simulink model "ASM_Traffic_MultiCore"  (R2026a)
settings: Solver=ode1  StartTime=SIM.tstart.v  StopTime=SIM.tend.v  FixedStep=SIM.StepSize.v
PostLoadFcn:
  | if any(exist('dsrtsu_mdlpostloadfcn', 'file') ~= 0), dsrtsu_mdlpostloadfcn('Execute', bdroot); end
  | try, asm_mdl_postloadfcn(bdroot, 'UpdateModel', 3600); catch, disp(lasterr); end,
InitFcn:
  | , if any(exist('rtifpga_mdlclblib', 'file') ~= 0), rtifpga_mdlclblib('Init', bdroot); end,
  | , if any(exist('dsmpb_private', 'file') ~= 0), dsmpb_private('dsmpb_mdlclblib', 'Init', bdroot); end,
model workspace (MAT data in the model file):
  asmReferencePath = [0 0.01 0.02 0.03 0.04 0.05 0.06 0.07 0.08 0.09 0.1 0.11 ... (350007 elements, 50001x7)]
  roadBounds : Simulink.Parameter (value not decoded)
  safetyAxes : Simulink.Parameter (value not decoded)
undefined symbols (not defined in the file): _to_, a0b2, ASM_BrakeHydraulics_DemoSystems, ASM_VehicleDynamics_DemoSystems, b98103fe8ad365046cd0, BrakeCircuit, controllerConfig, CPT, Crankshaft, DiscIntNeverNeededParam, dsmsi, FinalDriveAssembly, MDL, ModeSignals, mu, Pos_BrakePedal_Maneuver, rad, RefSignals, roadFamilyData, roadFamilyId, s_to_rpm, SIM, SoftECU, Suspension, Tire, Transmission
libraries: ASM_Traffic_lib x135, simulink x98, ASM_Utils_lib x77, ASM_VehicleDynamics_lib x70, ASM_Environment_lib x22, dsmpblib x20, dsmsilib x15, MDLD_Utils_lib x10, ASM_BrakeHydraulics_lib x3, sl_discontinuities x2
(part 57 of 65)

== system ASM_Traffic_MultiCore/Environment/GroundTruth/UserInterface/PAR_Plant/Fellow_Vehicles/Lightstates_Fellow3/Indicator_State[] ==
  Fellow_TurnLights[] : Inport
  ASM_OSI_Mapping : Subsystem
  Ext_Indicator_State[] : Constant  Value=0
  Multiport Switch : MultiPortSwitch  DataPortOrder=Zero-based contiguous  zeroidx=on  SaturateOnIntegerOverflow=off  InputSameDT=off
  Rounding Function : Rounding  Operator=round
  Saturation : Saturate  UpperLimit=2  LowerLimit=0
  Stim_Indicator_State[] : Constant  Value=0
  Sw_Indicator[0Stim|1Ext|2Mnv] : Constant  Value=2
  Indicator_State[] : Outport  VectorParamsAs1DForOutWhenUnconnected=off
  wires:
  ASM_OSI_Mapping/1(Indicator_State[]) -> Multiport Switch/4  "Mnv_Indicator_State[]"
  Stim_Indicator_State[]/1 -> Multiport Switch/2  "Stim_Indicator_State[]"
  Multiport Switch/1 -> Indicator_State[]/1  "Indicator_State[]"
  Saturation/1 -> Multiport Switch/1
  Rounding Function/1 -> Saturation/1
  Ext_Indicator_State[]/1 -> Multiport Switch/3  "Ext_Indicator_State[]"
  Fellow_TurnLights[]/1 -> ASM_OSI_Mapping/1(Fellow_TurnLights[])
  Sw_Indicator[0Stim|1Ext|2Mnv]/1 -> Rounding Function/1  "Sw_Indicator[0Stim|1Ext|2Mnv]"

== system ASM_Traffic_MultiCore/Environment/GroundTruth/UserInterface/PAR_Plant/Fellow_Vehicles/Lightstates_Fellow30/Indicator_State[] ==
  Fellow_TurnLights[] : Inport
  ASM_OSI_Mapping : Subsystem
  Ext_Indicator_State[] : Constant  Value=0
  Multiport Switch : MultiPortSwitch  DataPortOrder=Zero-based contiguous  zeroidx=on  SaturateOnIntegerOverflow=off  InputSameDT=off
  Rounding Function : Rounding  Operator=round
  Saturation : Saturate  UpperLimit=2  LowerLimit=0
  Stim_Indicator_State[] : Constant  Value=0
  Sw_Indicator[0Stim|1Ext|2Mnv] : Constant  Value=2
  Indicator_State[] : Outport  VectorParamsAs1DForOutWhenUnconnected=off
  wires:
  Sw_Indicator[0Stim|1Ext|2Mnv]/1 -> Rounding Function/1  "Sw_Indicator[0Stim|1Ext|2Mnv]"
  Fellow_TurnLights[]/1 -> ASM_OSI_Mapping/1(Fellow_TurnLights[])
  Ext_Indicator_State[]/1 -> Multiport Switch/3  "Ext_Indicator_State[]"
  Rounding Function/1 -> Saturation/1
  Saturation/1 -> Multiport Switch/1
  Multiport Switch/1 -> Indicator_State[]/1  "Indicator_State[]"
  Stim_Indicator_State[]/1 -> Multiport Switch/2  "Stim_Indicator_State[]"
  ASM_OSI_Mapping/1(Indicator_State[]) -> Multiport Switch/4  "Mnv_Indicator_State[]"

== system ASM_Traffic_MultiCore/Environment/GroundTruth/UserInterface/PAR_Plant/Fellow_Vehicles/Lightstates_Fellow4/Indicator_State[] ==
  Fellow_TurnLights[] : Inport
  ASM_OSI_Mapping : Subsystem
  Ext_Indicator_State[] : Constant  Value=0
  Multiport Switch : MultiPortSwitch  DataPortOrder=Zero-based contiguous  zeroidx=on  SaturateOnIntegerOverflow=off  InputSameDT=off
  Rounding Function : Rounding  Operator=round
  Saturation : Saturate  UpperLimit=2  LowerLimit=0
  Stim_Indicator_State[] : Constant  Value=0
  Sw_Indicator[0Stim|1Ext|2Mnv] : Constant  Value=2
  Indicator_State[] : Outport  VectorParamsAs1DForOutWhenUnconnected=off
  wires:
  Sw_Indicator[0Stim|1Ext|2Mnv]/1 -> Rounding Function/1  "Sw_Indicator[0Stim|1Ext|2Mnv]"
  Fellow_TurnLights[]/1 -> ASM_OSI_Mapping/1(Fellow_TurnLights[])
  Ext_Indicator_State[]/1 -> Multiport Switch/3  "Ext_Indicator_State[]"
  Rounding Function/1 -> Saturation/1
  Saturation/1 -> Multiport Switch/1
  Multiport Switch/1 -> Indicator_State[]/1  "Indicator_State[]"
  Stim_Indicator_State[]/1 -> Multiport Switch/2  "Stim_Indicator_State[]"
  ASM_OSI_Mapping/1(Indicator_State[]) -> Multiport Switch/4  "Mnv_Indicator_State[]"

== system ASM_Traffic_MultiCore/Environment/GroundTruth/UserInterface/PAR_Plant/Fellow_Vehicles/Lightstates_Fellow5/Indicator_State[] ==
  Fellow_TurnLights[] : Inport
  ASM_OSI_Mapping : Subsystem
  Ext_Indicator_State[] : Constant  Value=0
  Multiport Switch : MultiPortSwitch  DataPortOrder=Zero-based contiguous  zeroidx=on  SaturateOnIntegerOverflow=off  InputSameDT=off
  Rounding Function : Rounding  Operator=round
  Saturation : Saturate  UpperLimit=2  LowerLimit=0
  Stim_Indicator_State[] : Constant  Value=0
  Sw_Indicator[0Stim|1Ext|2Mnv] : Constant  Value=2
  Indicator_State[] : Outport  VectorParamsAs1DForOutWhenUnconnected=off
  wires:
  ASM_OSI_Mapping/1(Indicator_State[]) -> Multiport Switch/4  "Mnv_Indicator_State[]"
  Stim_Indicator_State[]/1 -> Multiport Switch/2  "Stim_Indicator_State[]"
  Multiport Switch/1 -> Indicator_State[]/1  "Indicator_State[]"
  Saturation/1 -> Multiport Switch/1
  Rounding Function/1 -> Saturation/1
  Ext_Indicator_State[]/1 -> Multiport Switch/3  "Ext_Indicator_State[]"
  Fellow_TurnLights[]/1 -> ASM_OSI_Mapping/1(Fellow_TurnLights[])
  Sw_Indicator[0Stim|1Ext|2Mnv]/1 -> Rounding Function/1  "Sw_Indicator[0Stim|1Ext|2Mnv]"

== system ASM_Traffic_MultiCore/Environment/GroundTruth/UserInterface/PAR_Plant/Fellow_Vehicles/Lightstates_Fellow6/Indicator_State[] ==
  Fellow_TurnLights[] : Inport
  ASM_OSI_Mapping : Subsystem
  Ext_Indicator_State[] : Constant  Value=0
  Multiport Switch : MultiPortSwitch  DataPortOrder=Zero-based contiguous  zeroidx=on  SaturateOnIntegerOverflow=off  InputSameDT=off
  Rounding Function : Rounding  Operator=round
  Saturation : Saturate  UpperLimit=2  LowerLimit=0
  Stim_Indicator_State[] : Constant  Value=0
  Sw_Indicator[0Stim|1Ext|2Mnv] : Constant  Value=2
  Indicator_State[] : Outport  VectorParamsAs1DForOutWhenUnconnected=off
  wires:
  Sw_Indicator[0Stim|1Ext|2Mnv]/1 -> Rounding Function/1  "Sw_Indicator[0Stim|1Ext|2Mnv]"
  Fellow_TurnLights[]/1 -> ASM_OSI_Mapping/1(Fellow_TurnLights[])
  Ext_Indicator_State[]/1 -> Multiport Switch/3  "Ext_Indicator_State[]"
  Rounding Function/1 -> Saturation/1
  Saturation/1 -> Multiport Switch/1
  Multiport Switch/1 -> Indicator_State[]/1  "Indicator_State[]"
  Stim_Indicator_State[]/1 -> Multiport Switch/2  "Stim_Indicator_State[]"
  ASM_OSI_Mapping/1(Indicator_State[]) -> Multiport Switch/4  "Mnv_Indicator_State[]"

== system ASM_Traffic_MultiCore/Environment/GroundTruth/UserInterface/PAR_Plant/Fellow_Vehicles/Lightstates_Fellow7/Indicator_State[] ==
  Fellow_TurnLights[] : Inport
  ASM_OSI_Mapping : Subsystem
  Ext_Indicator_State[] : Constant  Value=0
  Multiport Switch : MultiPortSwitch  DataPortOrder=Zero-based contiguous  zeroidx=on  SaturateOnIntegerOverflow=off  InputSameDT=off
  Rounding Function : Rounding  Operator=round
  Saturation : Saturate  UpperLimit=2  LowerLimit=0
  Stim_Indicator_State[] : Constant  Value=0
  Sw_Indicator[0Stim|1Ext|2Mnv] : Constant  Value=2
  Indicator_State[] : Outport  VectorParamsAs1DForOutWhenUnconnected=off
  wires:
  ASM_OSI_Mapping/1(Indicator_State[]) -> Multiport Switch/4  "Mnv_Indicator_State[]"
  Stim_Indicator_State[]/1 -> Multiport Switch/2  "Stim_Indicator_State[]"
  Multiport Switch/1 -> Indicator_State[]/1  "Indicator_State[]"
  Saturation/1 -> Multiport Switch/1
  Rounding Function/1 -> Saturation/1
  Ext_Indicator_State[]/1 -> Multiport Switch/3  "Ext_Indicator_State[]"
  Fellow_TurnLights[]/1 -> ASM_OSI_Mapping/1(Fellow_TurnLights[])
  Sw_Indicator[0Stim|1Ext|2Mnv]/1 -> Rounding Function/1  "Sw_Indicator[0Stim|1Ext|2Mnv]"

== system ASM_Traffic_MultiCore/Environment/GroundTruth/UserInterface/PAR_Plant/Fellow_Vehicles/Lightstates_Fellow8/Indicator_State[] ==
  Fellow_TurnLights[] : Inport
  ASM_OSI_Mapping : Subsystem
  Ext_Indicator_State[] : Constant  Value=0
  Multiport Switch : MultiPortSwitch  DataPortOrder=Zero-based contiguous  zeroidx=on  SaturateOnIntegerOverflow=off  InputSameDT=off
  Rounding Function : Rounding  Operator=round
  Saturation : Saturate  UpperLimit=2  LowerLimit=0
  Stim_Indicator_State[] : Constant  Value=0
  Sw_Indicator[0Stim|1Ext|2Mnv] : Constant  Value=2
  Indicator_State[] : Outport  VectorParamsAs1DForOutWhenUnconnected=off
  wires:
  Sw_Indicator[0Stim|1Ext|2Mnv]/1 -> Rounding Function/1  "Sw_Indicator[0Stim|1Ext|2Mnv]"
  Fellow_TurnLights[]/1 -> ASM_OSI_Mapping/1(Fellow_TurnLights[])
  Ext_Indicator_State[]/1 -> Multiport Switch/3  "Ext_Indicator_State[]"
  Rounding Function/1 -> Saturation/1
  Saturation/1 -> Multiport Switch/1
  Multiport Switch/1 -> Indicator_State[]/1  "Indicator_State[]"
  Stim_Indicator_State[]/1 -> Multiport Switch/2  "Stim_Indicator_State[]"
  ASM_OSI_Mapping/1(Indicator_State[]) -> Multiport Switch/4  "Mnv_Indicator_State[]"

== system ASM_Traffic_MultiCore/Environment/GroundTruth/UserInterface/PAR_Plant/Fellow_Vehicles/Lightstates_Fellow9/Indicator_State[] ==
  Fellow_TurnLights[] : Inport
  ASM_OSI_Mapping : Subsystem
  Ext_Indicator_State[] : Constant  Value=0
  Multiport Switch : MultiPortSwitch  DataPortOrder=Zero-based contiguous  zeroidx=on  SaturateOnIntegerOverflow=off  InputSameDT=off
  Rounding Function : Rounding  Operator=round
  Saturation : Saturate  UpperLimit=2  LowerLimit=0
  Stim_Indicator_State[] : Constant  Value=0
  Sw_Indicator[0Stim|1Ext|2Mnv] : Constant  Value=2
  Indicator_State[] : Outport  VectorParamsAs1DForOutWhenUnconnected=off
  wires:
  ASM_OSI_Mapping/1(Indicator_State[]) -> Multiport Switch/4  "Mnv_Indicator_State[]"
  Stim_Indicator_State[]/1 -> Multiport Switch/2  "Stim_Indicator_State[]"
  Multiport Switch/1 -> Indicator_State[]/1  "Indicator_State[]"
  Saturation/1 -> Multiport Switch/1
  Rounding Function/1 -> Saturation/1
  Ext_Indicator_State[]/1 -> Multiport Switch/3  "Ext_Indicator_State[]"
  Fellow_TurnLights[]/1 -> ASM_OSI_Mapping/1(Fellow_TurnLights[])
  Sw_Indicator[0Stim|1Ext|2Mnv]/1 -> Rounding Function/1  "Sw_Indicator[0Stim|1Ext|2Mnv]"

== system ASM_Traffic_MultiCore/Environment/GroundTruth/UserInterface/PAR_Plant/HostVehicle_Data_AutomatedDrivingFunction/AutomatedDrivingFunction_1/Mappings ==
  Driver_Override_ACC_Active_In[0Off|1On] : Inport
  Driver_Override_ACC_Reason[0NoOverride|1BrakePedal|2AccPedal] : Inport  Port=2
  ACC_State[1OFF|2Standby|3ON] : Inport  Port=3
  Compare To Constant : simulink/Logic and Bit Operations/Compare To Constant  relop===  const=1  OutDataTypeStr=boolean
  Data Type Conversion : DataTypeConversion  SaturateOnIntegerOverflow=off  RndMeth=Floor
  DriverOverride_Reason_Idx[0BrakePedal|1SteeringInput] : Constant  Value=0
  Multiport Switch1 : MultiPortSwitch  DataPortIndices={-2,-1,0,1,2,3}  DataPortForDefault=Additional data port  DiagnosticForDefault=None  SaturateOnIntegerOverflow=off  InputSameDT=off
  Off : Constant  Value=0
  State_Active : Constant  Value=6
  State_Available : Constant  Value=4
  State_Other : Constant
  State_Standby : Constant  Value=5
  Switch1 : Switch  Criteria=u2 > Threshold  SaturateOnIntegerOverflow=off  InputSameDT=off
  Driver_Override_ACC_Active[0Off|1On] : Outport
  DriverOverride_Reason_Idx[] : Outport  Port=2
  State_Idx[] : Outport  Port=3
  wires:
  Driver_Override_ACC_Reason[0NoOverride|1BrakePedal|2AccPedal]/1 -> Compare To Constant/1
  Compare To Constant/1 -> Switch1/2
  ACC_State[1OFF|2Standby|3ON]/1 -> Multiport Switch1/1
  Multiport Switch1/1 -> State_Idx[]/1
  State_Standby/1 -> Multiport Switch1/3
  State_Available/1 -> Multiport Switch1/2
  State_Active/1 -> Multiport Switch1/4
  State_Other/1 -> Multiport Switch1/5
  Driver_Override_ACC_Active_In[0Off|1On]/1 -> Data Type Conversion/1
  Data Type Conversion/1 -> Switch1/1
  Off/1 -> Switch1/3
  Switch1/1 -> Driver_Override_ACC_Active[0Off|1On]/1
  DriverOverride_Reason_Idx[0BrakePedal|1SteeringInput]/1 -> DriverOverride_Reason_Idx[]/1

== system ASM_Traffic_MultiCore/Environment/GroundTruth/UserInterface/PAR_Plant/HostVehicle_Data_AutomatedDrivingFunction/AutomatedDrivingFunction_2/Mappings ==
  Driver_Override_ACC_Active_In[0Off|1On] : Inport
  Driver_Override_ACC_Reason[0NoOverride|1BrakePedal|2AccPedal] : Inport  Port=2
  AEB[0|1] : Inport  Port=3
  Compare To Constant : simulink/Logic and Bit Operations/Compare To Constant  relop===  const=1  OutDataTypeStr=boolean
  Data Type Conversion : DataTypeConversion  SaturateOnIntegerOverflow=off  RndMeth=Floor
  DriverOverride_Reason_Idx[0BrakePedal|1SteeringInput] : Constant  Value=0
  Multiport Switch1 : MultiPortSwitch  DataPortOrder=Zero-based contiguous  Inputs=2  DataPortIndices={-2,-1,0,1,2,3}  DataPortForDefault=Additional data port  DiagnosticForDefault=None  zeroidx=on  SaturateOnIntegerOverflow=off  InputSameDT=off
  Off : Constant  Value=0
  State_Active : Constant  Value=6
  State_Available : Constant  Value=4
  State_Other : Constant
  Switch1 : Switch  Criteria=u2 > Threshold  SaturateOnIntegerOverflow=off  InputSameDT=off
  Driver_Override_ACC_Active[0Off|1On] : Outport
  DriverOverride_Reason_Idx[] : Outport  Port=2
  State_Idx[] : Outport  Port=3
  wires:
  DriverOverride_Reason_Idx[0BrakePedal|1SteeringInput]/1 -> DriverOverride_Reason_Idx[]/1
  Driver_Override_ACC_Reason[0NoOverride|1BrakePedal|2AccPedal]/1 -> Compare To Constant/1
  AEB[0|1]/1 -> Multiport Switch1/1
  Multiport Switch1/1 -> State_Idx[]/1
  State_Active/1 -> Multiport Switch1/3
  State_Available/1 -> Multiport Switch1/2
  State_Other/1 -> Multiport Switch1/4
  Driver_Override_ACC_Active_In[0Off|1On]/1 -> Data Type Conversion/1
  Off/1 -> Switch1/3
  Compare To Constant/1 -> Switch1/2
  Data Type Conversion/1 -> Switch1/1
  Switch1/1 -> Driver_Override_ACC_Active[0Off|1On]/1

== system ASM_Traffic_MultiCore/Environment/GroundTruth/UserInterface/PAR_Plant/HostVehicle_Data_AutomatedDrivingFunction/AutomatedDrivingFunction_3/Mappings ==
  Driver_Override_ACC_Active_In[0Off|1On] : Inport
  Driver_Override_ACC_Reason[0NoOverride|1BrakePedal|2AccPedal] : Inport  Port=2
  FCW[0|1] : Inport  Port=3
  Compare To Constant : simulink/Logic and Bit Operations/Compare To Constant  relop===  const=1  OutDataTypeStr=boolean
  Data Type Conversion : DataTypeConversion  SaturateOnIntegerOverflow=off  RndMeth=Floor
  DriverOverride_Reason_Idx[0BrakePedal|1SteeringInput] : Constant  Value=0
  Multiport Switch1 : MultiPortSwitch  DataPortOrder=Zero-based contiguous  Inputs=2  DataPortIndices={-2,-1,0,1,2,3}  DataPortForDefault=Additional data port  DiagnosticForDefault=None  zeroidx=on  SaturateOnIntegerOverflow=off  InputSameDT=off
  Off : Constant  Value=0
  State_Active : Constant  Value=6
  State_Available : Constant  Value=4
  State_Other : Constant
  Switch1 : Switch  Criteria=u2 > Threshold  SaturateOnIntegerOverflow=off  InputSameDT=off
  Driver_Override_ACC_Active[0Off|1On] : Outport
  DriverOverride_Reason_Idx[] : Outport  Port=2
  State_Idx[] : Outport  Port=3
  wires:
  Driver_Override_ACC_Reason[0NoOverride|1BrakePedal|2AccPedal]/1 -> Compare To Constant/1
  FCW[0|1]/1 -> Multiport Switch1/1
  Multiport Switch1/1 -> State_Idx[]/1
  State_Active/1 -> Multiport Switch1/3
  State_Available/1 -> Multiport Switch1/2
  State_Other/1 -> Multiport Switch1/4
  Driver_Override_ACC_Active_In[0Off|1On]/1 -> Data Type Conversion/1
  Off/1 -> Switch1/3
  Switch1/1 -> Driver_Override_ACC_Active[0Off|1On]/1
  Data Type Conversion/1 -> Switch1/1
  Compare To Constant/1 -> Switch1/2
  DriverOverride_Reason_Idx[0BrakePedal|1SteeringInput]/1 -> DriverOverride_Reason_Idx[]/1

== system ASM_Traffic_MultiCore/Environment/Road/UserInterface/PAR_Plant/Objects_DataStreams/DataStream_1/TrafficLight1_Control ==
  Reset[] : Inport
  1-D Lookup Table : Lookup_n-D  NumberOfTableDimensions=1  BreakpointsForDimension1=MDL.Traffic.TrafficLight_Control.Map_TrafficLight1.x  Table=MDL.Traffic.TrafficLight_Control.Map_TrafficLight1.v  InterpMethod=Nearest  InternalRulePriority=Speed  RndMeth=Simplest
  Detect Increase : simulink/Logic and Bit Operations/Detect Increase  vinit=0.0  OutDataTypeStr=boolean
  Detect Increase1 : simulink/Logic and Bit Operations/Detect Increase  vinit=0.0  OutDataTypeStr=boolean
  Discrete-Time Integrator : DiscreteIntegrator  ExternalReset=rising  SampleTime=-1  ICPrevOutput=DiscIntNeverNeededParam  ICPrevScaledInput=DiscIntNeverNeededParam
  Integrant : Constant
  Logical Operator : Logic  Operator=OR  AllPortsSameDT=off  OutDataTypeStr=boolean
  Relational Operator : RelationalOperator  Operator=<  OutDataTypeStr=boolean  InputSameDT=off
  TrafficLightPeriod[s] : Constant  Value=MDL.Traffic.TrafficLight_Control.Map_TrafficLight3.x(end)
  Unit Delay : UnitDelay  SampleTime=-1
  TrafficLightState[1|2|3|4] : Outport  VectorParamsAs1DForOutWhenUnconnected=off
  wires:
  Detect Increase1/1 -> Logical Operator/1
  Detect Increase/1 -> Logical Operator/2
  Logical Operator/1 -> Discrete-Time Integrator/2
  Reset[]/1 -> Detect Increase1/1
  1-D Lookup Table/1 -> TrafficLightState[1|2|3|4]/1  "TrafficLight1_State[1Red|2Yellow|3RedYellow|4Green]"
  TrafficLightPeriod[s]/1 -> Relational Operator/1
  Integrant/1 -> Discrete-Time Integrator/1
  Relational Operator/1 -> Detect Increase/1
  Discrete-Time Integrator/1 -> Unit Delay/1, 1-D Lookup Table/1
  Unit Delay/1 -> Relational Operator/2

== system ASM_Traffic_MultiCore/Environment/Road/UserInterface/PAR_Plant/Objects_DataStreams/DataStream_2/TrafficLight2_Control ==
  Reset[] : Inport
  1-D Lookup Table : Lookup_n-D  NumberOfTableDimensions=1  BreakpointsForDimension1=MDL.Traffic.TrafficLight_Control.Map_TrafficLight2.x  Table=MDL.Traffic.TrafficLight_Control.Map_TrafficLight2.v  InterpMethod=Nearest  InternalRulePriority=Speed  RndMeth=Simplest
  Detect Increase : simulink/Logic and Bit Operations/Detect Increase  vinit=0.0  OutDataTypeStr=boolean
  Detect Increase1 : simulink/Logic and Bit Operations/Detect Increase  vinit=0.0  OutDataTypeStr=boolean
  Discrete-Time Integrator : DiscreteIntegrator  ExternalReset=rising  SampleTime=-1  ICPrevOutput=DiscIntNeverNeededParam  ICPrevScaledInput=DiscIntNeverNeededParam
  Integrant : Constant
  Logical Operator : Logic  Operator=OR  AllPortsSameDT=off  OutDataTypeStr=boolean
  Relational Operator : RelationalOperator  Operator=<  OutDataTypeStr=boolean  InputSameDT=off
  TrafficLightPeriod[s] : Constant  Value=MDL.Traffic.TrafficLight_Control.Map_TrafficLight2.x(end)
  Unit Delay : UnitDelay  SampleTime=-1
  TrafficLightState[1|2|3|4] : Outport  VectorParamsAs1DForOutWhenUnconnected=off
  wires:
  Detect Increase1/1 -> Logical Operator/1
  Detect Increase/1 -> Logical Operator/2
  Logical Operator/1 -> Discrete-Time Integrator/2
  Reset[]/1 -> Detect Increase1/1
  1-D Lookup Table/1 -> TrafficLightState[1|2|3|4]/1  "TrafficLight2_State[1Red|2Yellow|3RedYellow|4Green]"
  TrafficLightPeriod[s]/1 -> Relational Operator/1
  Integrant/1 -> Discrete-Time Integrator/1
  Relational Operator/1 -> Detect Increase/1
  Discrete-Time Integrator/1 -> Unit Delay/1, 1-D Lookup Table/1
  Unit Delay/1 -> Relational Operator/2

== system ASM_Traffic_MultiCore/Environment/Road/UserInterface/PAR_Plant/Objects_DataStreams/DataStream_3/TrafficLight3_Control ==
  Reset[] : Inport
  1-D Lookup Table : Lookup_n-D  NumberOfTableDimensions=1  BreakpointsForDimension1=MDL.Traffic.TrafficLight_Control.Map_TrafficLight3.x  Table=MDL.Traffic.TrafficLight_Control.Map_TrafficLight3.v  InterpMethod=Nearest  InternalRulePriority=Speed  RndMeth=Simplest
  Detect Increase : simulink/Logic and Bit Operations/Detect Increase  vinit=0.0  OutDataTypeStr=boolean
  Detect Increase1 : simulink/Logic and Bit Operations/Detect Increase  vinit=0.0  OutDataTypeStr=boolean
  Discrete-Time Integrator : DiscreteIntegrator  ExternalReset=rising  SampleTime=-1  ICPrevOutput=DiscIntNeverNeededParam  ICPrevScaledInput=DiscIntNeverNeededParam
  Integrant : Constant
  Logical Operator : Logic  Operator=OR  AllPortsSameDT=off  OutDataTypeStr=boolean
  Relational Operator : RelationalOperator  Operator=<  OutDataTypeStr=boolean  InputSameDT=off
  TrafficLightPeriod[s] : Constant  Value=MDL.Traffic.TrafficLight_Control.Map_TrafficLight2.x(end)
  Unit Delay : UnitDelay  SampleTime=-1
  TrafficLightState[1|2|3|4] : Outport  VectorParamsAs1DForOutWhenUnconnected=off
  wires:
  Unit Delay/1 -> Relational Operator/2
  Discrete-Time Integrator/1 -> 1-D Lookup Table/1, Unit Delay/1
  Relational Operator/1 -> Detect Increase/1
  Integrant/1 -> Discrete-Time Integrator/1
  TrafficLightPeriod[s]/1 -> Relational Operator/1
  1-D Lookup Table/1 -> TrafficLightState[1|2|3|4]/1  "TrafficLight3_State[1Red|2Yellow|3RedYellow|4Green]"
  Reset[]/1 -> Detect Increase1/1
  Logical Operator/1 -> Discrete-Time Integrator/2
  Detect Increase/1 -> Logical Operator/2
  Detect Increase1/1 -> Logical Operator/1

== system ASM_Traffic_MultiCore/Environment/Road/UserInterface/PAR_Plant/Objects_DataStreams/DataStream_4/TrafficLight4_Control ==
  Reset[] : Inport
  1-D Lookup Table : Lookup_n-D  NumberOfTableDimensions=1  BreakpointsForDimension1=MDL.Traffic.TrafficLight_Control.Map_TrafficLight4.x  Table=MDL.Traffic.TrafficLight_Control.Map_TrafficLight4.v  InterpMethod=Nearest  InternalRulePriority=Speed  RndMeth=Simplest
  Detect Increase : simulink/Logic and Bit Operations/Detect Increase  vinit=0.0  OutDataTypeStr=boolean
  Detect Increase1 : simulink/Logic and Bit Operations/Detect Increase  vinit=0.0  OutDataTypeStr=boolean
  Discrete-Time Integrator : DiscreteIntegrator  ExternalReset=rising  SampleTime=-1  ICPrevOutput=DiscIntNeverNeededParam  ICPrevScaledInput=DiscIntNeverNeededParam
  Integrant : Constant
  Logical Operator : Logic  Operator=OR  AllPortsSameDT=off  OutDataTypeStr=boolean
  Relational Operator : RelationalOperator  Operator=<  OutDataTypeStr=boolean  InputSameDT=off
  TrafficLightPeriod[s] : Constant  Value=MDL.Traffic.TrafficLight_Control.Map_TrafficLight2.x(end)
  Unit Delay : UnitDelay  SampleTime=-1
  TrafficLightState[1|2|3|4] : Outport  VectorParamsAs1DForOutWhenUnconnected=off
  wires:
  Detect Increase1/1 -> Logical Operator/1
  Detect Increase/1 -> Logical Operator/2
  Logical Operator/1 -> Discrete-Time Integrator/2
  Reset[]/1 -> Detect Increase1/1
  1-D Lookup Table/1 -> TrafficLightState[1|2|3|4]/1  "TrafficLight4_State[1Red|2Yellow|3RedYellow|4Green]"
  TrafficLightPeriod[s]/1 -> Relational Operator/1
  Integrant/1 -> Discrete-Time Integrator/1
  Relational Operator/1 -> Detect Increase/1
  Discrete-Time Integrator/1 -> Unit Delay/1, 1-D Lookup Table/1
  Unit Delay/1 -> Relational Operator/2

== system ASM_Traffic_MultiCore/Environment/Road/UserInterface/PAR_Plant/Objects_DataStreams/DataStream_5/avoid_incomplete_trace2source ==
  In1 : Inport
  DummyGain : Gain
  Out1 : Outport
  wires:
  In1/1 -> DummyGain/1
  DummyGain/1 -> Out1/1

== system ASM_Traffic_MultiCore/Environment/Road/UserInterface/PAR_Plant/Objects_DataStreams/DataStream_6/avoid_incomplete_trace2source ==
  In1 : Inport
  DummyGain : Gain
  Out1 : Outport
  wires:
  In1/1 -> DummyGain/1
  DummyGain/1 -> Out1/1

== system ASM_Traffic_MultiCore/Environment/Road/UserInterface/PAR_Plant/Objects_DataStreams/DataStream_7/avoid_incomplete_trace2source ==
  In1 : Inport
  DummyGain : Gain
  Out1 : Outport
  wires:
  In1/1 -> DummyGain/1
  DummyGain/1 -> Out1/1

== system ASM_Traffic_MultiCore/Environment/Road/UserInterface/PAR_Plant/Objects_DataStreams/DataStream_8/avoid_incomplete_trace2source ==
  In1 : Inport
  DummyGain : Gain
  Out1 : Outport
  wires:
  In1/1 -> DummyGain/1
  DummyGain/1 -> Out1/1

== system ASM_Traffic_MultiCore/Environment/Sensors/PlantModel/Object_Sensor_2D/ObjectData/Sensor1/ASMSignalCollector ==
  Object_Positions : Inport
  Object_Properties_Box : Inport  Port=2
  Object_Custom_Values : Inport  Port=3
  Bus Creator1 : BusCreator  Inputs=3
  Bus Selector : BusSelector  OutputSignals=Object_Positions
  Bus Selector1 : BusSelector  OutputSignals=Object_Properties_Box
  ASMSignalBus : Outport  VectorParamsAs1DForOutWhenUnconnected=off
  wires:
  Object_Positions/1 -> Bus Selector/1
  Object_Custom_Values/1 -> Bus Creator1/3
  Bus Creator1/1 -> ASMSignalBus/1  "ObjectData"
  Object_Properties_Box/1 -> Bus Selector1/1
  Bus Selector/1 -> Bus Creator1/1  "<Object_Positions>"
  Bus Selector1/1 -> Bus Creator1/2  "<Object_Properties_Box>"

== system ASM_Traffic_MultiCore/Environment/Sensors/PlantModel/Object_Sensor_2D/ObjectData/Sensor1/GetFellowPositionVector ==
  <FellowPositions> : Inport
  Bus Selector11 : BusSelector  OutputSignals=Pos_Fellows_MainPnt_CoorSys_E[x;y;z][m].Pos_x_Fellows[m],Pos_Fellows_MainPnt_CoorSys_E[x;y;z][m].Pos_y_Fellows[m],Pos_Fellows_MainPnt_CoorSys_E[x;y;z][m].Pos_z_Fellows[m],Angle_Fellows[x;y;z][deg].Angle_Roll_Fellows[deg],Angle_Fellows[x;y;z][deg].Angle_Pitch_Fellows[deg],Angle_Fellows[x;y;z][deg].Angle_Yaw_Fellows[deg]
  Mux1 : Mux  Inputs=3
  Mux2 : Mux  Inputs=3
  Pos_Fellows_MainPnt_CoorSys_E[x;y;z][m] : Outport  VectorParamsAs1DForOutWhenUnconnected=off
  Angle_Fellows[deg] : Outport  Port=2  VectorParamsAs1DForOutWhenUnconnected=off
  wires:
  Mux2/1 -> Pos_Fellows_MainPnt_CoorSys_E[x;y;z][m]/1  "Pos_Fellows_MainPnt_CoorSys_E[x;y;z][m]"
  Mux1/1 -> Angle_Fellows[deg]/1  "Pos_Fellows_MainPnt_CoorSys_E_vec"
  Bus Selector11/4 -> Mux1/1  "<Angle_Roll_Fellows[deg]>"
  Bus Selector11/1 -> Mux2/1  "<Pos_x_Fellows[m]>"
  Bus Selector11/2 -> Mux2/2  "<Pos_y_Fellows[m]>"
  Bus Selector11/6 -> Mux1/3  "<Angle_Yaw_Fellows[deg]>"
  Bus Selector11/5 -> Mux1/2  "<Angle_Pitch_Fellows[deg]>"
  <FellowPositions>/1 -> Bus Selector11/1
  Bus Selector11/3 -> Mux2/3  "<Pos_z_Fellows[m]>"

== system ASM_Traffic_MultiCore/Environment/Sensors/PlantModel/Object_Sensor_2D/ObjectData/Sensor1/Object_Custom_Values ==
  TrafficObject_Type[] : Inport
  TrafficObject_Type_Data[] : Inport  Port=2
  CUSTOM_SENSOR_OUTPUT : ASM_Traffic_lib/Sensors/Custom_Sensor/CUSTOM_SENSOR_OUTPUT  Tag=ASM_SUBCOMPONENT  ASMProperties=struct('Name','CUSTOM_SENSOR_OUTPUT','Version','5.0','Library','ASM_Traffic_lib')  ASMInstanceName=custom_sensor_output  ASMInstanceID=11
      settings: AttributesFormatString=Instance Name: %<ASMInstanceName>\nInstance ID: %<ASMInstanceID>
  CUSTOM_SENSOR_OUTPUT1 : ASM_Traffic_lib/Sensors/Custom_Sensor/CUSTOM_SENSOR_OUTPUT  Tag=ASM_SUBCOMPONENT  ASMProperties=struct('Name','CUSTOM_SENSOR_OUTPUT','Version','5.0','Library','ASM_Traffic_lib')  ASMInstanceName=custom_sensor_output  ASMInstanceID=12
      settings: AttributesFormatString=Instance Name: %<ASMInstanceName>\nInstance ID: %<ASMInstanceID>
  CUSTOM_SENSOR_OUTPUT2 : ASM_Traffic_lib/Sensors/Custom_Sensor/CUSTOM_SENSOR_OUTPUT  Tag=ASM_SUBCOMPONENT  ASMProperties=struct('Name','CUSTOM_SENSOR_OUTPUT','Version','5.0','Library','ASM_Traffic_lib')  ASMInstanceName=custom_sensor_output  ASMInstanceID=13
      settings: AttributesFormatString=Instance Name: %<ASMInstanceName>\nInstance ID: %<ASMInstanceID>
  Terminator : Terminator
  Terminator1 : Terminator
  Terminator2 : Terminator
  Vectorize_Signals : Subsystem
  "[11:15]" : Selector  IndexOptions=Index vector (dialog)  Indices=[11:15]  OutputSizes=1
  "[1:5]" : Selector  IndexOptions=Index vector (dialog)  Indices=[1:5]  OutputSizes=1
  "[6:10]" : Selector  IndexOptions=Index vector (dialog)  Indices=[6:10]  OutputSizes=1
  Object_Custom_Values[] : Outport  VectorParamsAs1DForOutWhenUnconnected=off
  wires:
  CUSTOM_SENSOR_OUTPUT2/2 -> Vectorize_Signals/3(SensorOutput3)
  CUSTOM_SENSOR_OUTPUT1/2 -> Vectorize_Signals/2(SensorOutput2)
  Vectorize_Signals/1(Vectorized_Custom_Values) -> Object_Custom_Values[]/1
  CUSTOM_SENSOR_OUTPUT/2 -> Vectorize_Signals/1(SensorOutput1)
  CUSTOM_SENSOR_OUTPUT2/1 -> Terminator2/1
  CUSTOM_SENSOR_OUTPUT1/1 -> Terminator1/1
  CUSTOM_SENSOR_OUTPUT/1 -> Terminator/1
  "[6:10]"/1 -> CUSTOM_SENSOR_OUTPUT1/1
  TrafficObject_Type[]/1 -> "[11:15]"/1, "[6:10]"/1, "[1:5]"/1
  TrafficObject_Type_Data[]/1 -> CUSTOM_SENSOR_OUTPUT2/2, CUSTOM_SENSOR_OUTPUT1/2, CUSTOM_SENSOR_OUTPUT/2
  "[1:5]"/1 -> CUSTOM_SENSOR_OUTPUT/1
  "[11:15]"/1 -> CUSTOM_SENSOR_OUTPUT2/1

== system ASM_Traffic_MultiCore/Environment/Sensors/PlantModel/Object_Sensor_2D/ObjectData/Sensor2/ASMSignalCollector ==
  Object_Positions : Inport
  Object_Properties_Box : Inport  Port=2
  Object_Custom_Values : Inport  Port=3
  Bus Creator1 : BusCreator  Inputs=3
  Bus Selector : BusSelector  OutputSignals=Object_Positions
  Bus Selector1 : BusSelector  OutputSignals=Object_Properties_Box
  ASMSignalBus : Outport  VectorParamsAs1DForOutWhenUnconnected=off
  wires:
  Object_Positions/1 -> Bus Selector/1
  Object_Custom_Values/1 -> Bus Creator1/3
  Bus Creator1/1 -> ASMSignalBus/1  "ObjectData"
  Object_Properties_Box/1 -> Bus Selector1/1
  Bus Selector/1 -> Bus Creator1/1  "<Object_Positions>"
  Bus Selector1/1 -> Bus Creator1/2  "<Object_Properties_Box>"

== system ASM_Traffic_MultiCore/Environment/Sensors/PlantModel/Object_Sensor_2D/ObjectData/Sensor2/GetFellowPositionVector ==
  <FellowPositions> : Inport
  Bus Selector11 : BusSelector  OutputSignals=Pos_Fellows_MainPnt_CoorSys_E[x;y;z][m].Pos_x_Fellows[m],Pos_Fellows_MainPnt_CoorSys_E[x;y;z][m].Pos_y_Fellows[m],Pos_Fellows_MainPnt_CoorSys_E[x;y;z][m].Pos_z_Fellows[m],Angle_Fellows[x;y;z][deg].Angle_Roll_Fellows[deg],Angle_Fellows[x;y;z][deg].Angle_Pitch_Fellows[deg],Angle_Fellows[x;y;z][deg].Angle_Yaw_Fellows[deg]
  Mux1 : Mux  Inputs=3
  Mux2 : Mux  Inputs=3
  Pos_Fellows_MainPnt_CoorSys_E[x;y;z][m] : Outport  VectorParamsAs1DForOutWhenUnconnected=off
  Angle_Fellows[deg] : Outport  Port=2  VectorParamsAs1DForOutWhenUnconnected=off
  wires:
  Mux2/1 -> Pos_Fellows_MainPnt_CoorSys_E[x;y;z][m]/1  "Pos_Fellows_MainPnt_CoorSys_E[x;y;z][m]"
  Mux1/1 -> Angle_Fellows[deg]/1  "Pos_Fellows_MainPnt_CoorSys_E_vec"
  Bus Selector11/4 -> Mux1/1  "<Angle_Roll_Fellows[deg]>"
  Bus Selector11/1 -> Mux2/1  "<Pos_x_Fellows[m]>"
  Bus Selector11/2 -> Mux2/2  "<Pos_y_Fellows[m]>"
  Bus Selector11/6 -> Mux1/3  "<Angle_Yaw_Fellows[deg]>"
  Bus Selector11/5 -> Mux1/2  "<Angle_Pitch_Fellows[deg]>"
  <FellowPositions>/1 -> Bus Selector11/1
  Bus Selector11/3 -> Mux2/3  "<Pos_z_Fellows[m]>"

== system ASM_Traffic_MultiCore/Environment/Sensors/PlantModel/Object_Sensor_2D/ObjectData/Sensor2/Object_Custom_Values ==
  TrafficObject_Type[] : Inport
  TrafficObject_Type_Data[] : Inport  Port=2
  CUSTOM_SENSOR_OUTPUT : ASM_Traffic_lib/Sensors/Custom_Sensor/CUSTOM_SENSOR_OUTPUT  Tag=ASM_SUBCOMPONENT  ASMProperties=struct('Name','CUSTOM_SENSOR_OUTPUT','Version','5.0','Library','ASM_Traffic_lib')  ASMInstanceName=custom_sensor_output  ASMInstanceID=14
      settings: AttributesFormatString=Instance Name: %<ASMInstanceName>\nInstance ID: %<ASMInstanceID>
  CUSTOM_SENSOR_OUTPUT1 : ASM_Traffic_lib/Sensors/Custom_Sensor/CUSTOM_SENSOR_OUTPUT  Tag=ASM_SUBCOMPONENT  ASMProperties=struct('Name','CUSTOM_SENSOR_OUTPUT','Version','5.0','Library','ASM_Traffic_lib')  ASMInstanceName=custom_sensor_output  ASMInstanceID=15
      settings: AttributesFormatString=Instance Name: %<ASMInstanceName>\nInstance ID: %<ASMInstanceID>
  CUSTOM_SENSOR_OUTPUT2 : ASM_Traffic_lib/Sensors/Custom_Sensor/CUSTOM_SENSOR_OUTPUT  Tag=ASM_SUBCOMPONENT  ASMProperties=struct('Name','CUSTOM_SENSOR_OUTPUT','Version','5.0','Library','ASM_Traffic_lib')  ASMInstanceName=custom_sensor_output  ASMInstanceID=16
      settings: AttributesFormatString=Instance Name: %<ASMInstanceName>\nInstance ID: %<ASMInstanceID>
  Terminator : Terminator
  Terminator1 : Terminator
  Terminator2 : Terminator
  Vectorize_Signals : Subsystem
  "[11:15]" : Selector  IndexOptions=Index vector (dialog)  Indices=[11:15]  OutputSizes=1
  "[1:5]" : Selector  IndexOptions=Index vector (dialog)  Indices=[1:5]  OutputSizes=1
  "[6:10]" : Selector  IndexOptions=Index vector (dialog)  Indices=[6:10]  OutputSizes=1
  Object_Custom_Values[] : Outport  VectorParamsAs1DForOutWhenUnconnected=off
  wires:
  "[11:15]"/1 -> CUSTOM_SENSOR_OUTPUT2/1
  "[1:5]"/1 -> CUSTOM_SENSOR_OUTPUT/1
  TrafficObject_Type_Data[]/1 -> CUSTOM_SENSOR_OUTPUT1/2, CUSTOM_SENSOR_OUTPUT2/2, CUSTOM_SENSOR_OUTPUT/2
  TrafficObject_Type[]/1 -> "[11:15]"/1, "[6:10]"/1, "[1:5]"/1
  "[6:10]"/1 -> CUSTOM_SENSOR_OUTPUT1/1
  CUSTOM_SENSOR_OUTPUT/1 -> Terminator/1
  CUSTOM_SENSOR_OUTPUT1/1 -> Terminator1/1
  CUSTOM_SENSOR_OUTPUT2/1 -> Terminator2/1
  CUSTOM_SENSOR_OUTPUT/2 -> Vectorize_Signals/1(SensorOutput1)
  Vectorize_Signals/1(Vectorized_Custom_Values) -> Object_Custom_Values[]/1
  CUSTOM_SENSOR_OUTPUT1/2 -> Vectorize_Signals/2(SensorOutput2)
  CUSTOM_SENSOR_OUTPUT2/2 -> Vectorize_Signals/3(SensorOutput3)

== system ASM_Traffic_MultiCore/Environment/Sensors/PlantModel/Object_Sensor_2D/ObjectData/Sensor3/ASMSignalCollector ==
  Object_Positions : Inport
  Object_Properties_Box : Inport  Port=2
  Object_Custom_Values : Inport  Port=3
  Bus Creator1 : BusCreator  Inputs=3
  Bus Selector : BusSelector  OutputSignals=Object_Positions
  Bus Selector1 : BusSelector  OutputSignals=Object_Properties_Box
  ASMSignalBus : Outport  VectorParamsAs1DForOutWhenUnconnected=off
  wires:
  Object_Positions/1 -> Bus Selector/1
  Object_Custom_Values/1 -> Bus Creator1/3
  Bus Creator1/1 -> ASMSignalBus/1  "ObjectData"
  Object_Properties_Box/1 -> Bus Selector1/1
  Bus Selector/1 -> Bus Creator1/1  "<Object_Positions>"
  Bus Selector1/1 -> Bus Creator1/2  "<Object_Properties_Box>"

== system ASM_Traffic_MultiCore/Environment/Sensors/PlantModel/Object_Sensor_2D/ObjectData/Sensor3/GetFellowPositionVector ==
  <FellowPositions> : Inport
  Bus Selector11 : BusSelector  OutputSignals=Pos_Fellows_MainPnt_CoorSys_E[x;y;z][m].Pos_x_Fellows[m],Pos_Fellows_MainPnt_CoorSys_E[x;y;z][m].Pos_y_Fellows[m],Pos_Fellows_MainPnt_CoorSys_E[x;y;z][m].Pos_z_Fellows[m],Angle_Fellows[x;y;z][deg].Angle_Roll_Fellows[deg],Angle_Fellows[x;y;z][deg].Angle_Pitch_Fellows[deg],Angle_Fellows[x;y;z][deg].Angle_Yaw_Fellows[deg]
  Mux1 : Mux  Inputs=3
  Mux2 : Mux  Inputs=3
  Pos_Fellows_MainPnt_CoorSys_E[x;y;z][m] : Outport  VectorParamsAs1DForOutWhenUnconnected=off
  Angle_Fellows[deg] : Outport  Port=2  VectorParamsAs1DForOutWhenUnconnected=off
  wires:
  Mux2/1 -> Pos_Fellows_MainPnt_CoorSys_E[x;y;z][m]/1  "Pos_Fellows_MainPnt_CoorSys_E[x;y;z][m]"
  Mux1/1 -> Angle_Fellows[deg]/1  "Pos_Fellows_MainPnt_CoorSys_E_vec"
  Bus Selector11/4 -> Mux1/1  "<Angle_Roll_Fellows[deg]>"
  Bus Selector11/1 -> Mux2/1  "<Pos_x_Fellows[m]>"
  Bus Selector11/2 -> Mux2/2  "<Pos_y_Fellows[m]>"
  Bus Selector11/6 -> Mux1/3  "<Angle_Yaw_Fellows[deg]>"
  Bus Selector11/5 -> Mux1/2  "<Angle_Pitch_Fellows[deg]>"
  <FellowPositions>/1 -> Bus Selector11/1
  Bus Selector11/3 -> Mux2/3  "<Pos_z_Fellows[m]>"

== system ASM_Traffic_MultiCore/Environment/Sensors/PlantModel/Object_Sensor_2D/ObjectData/Sensor3/Object_Custom_Values ==
  TrafficObject_Type[] : Inport
  TrafficObject_Type_Data[] : Inport  Port=2
  CUSTOM_SENSOR_OUTPUT : ASM_Traffic_lib/Sensors/Custom_Sensor/CUSTOM_SENSOR_OUTPUT  Tag=ASM_SUBCOMPONENT  ASMProperties=struct('Name','CUSTOM_SENSOR_OUTPUT','Version','5.0','Library','ASM_Traffic_lib')  ASMInstanceName=custom_sensor_output  ASMInstanceID=17
      settings: AttributesFormatString=Instance Name: %<ASMInstanceName>\nInstance ID: %<ASMInstanceID>
  CUSTOM_SENSOR_OUTPUT1 : ASM_Traffic_lib/Sensors/Custom_Sensor/CUSTOM_SENSOR_OUTPUT  Tag=ASM_SUBCOMPONENT  ASMProperties=struct('Name','CUSTOM_SENSOR_OUTPUT','Version','5.0','Library','ASM_Traffic_lib')  ASMInstanceName=custom_sensor_output  ASMInstanceID=18
      settings: AttributesFormatString=Instance Name: %<ASMInstanceName>\nInstance ID: %<ASMInstanceID>
  CUSTOM_SENSOR_OUTPUT2 : ASM_Traffic_lib/Sensors/Custom_Sensor/CUSTOM_SENSOR_OUTPUT  Tag=ASM_SUBCOMPONENT  ASMProperties=struct('Name','CUSTOM_SENSOR_OUTPUT','Version','5.0','Library','ASM_Traffic_lib')  ASMInstanceName=custom_sensor_output  ASMInstanceID=19
      settings: AttributesFormatString=Instance Name: %<ASMInstanceName>\nInstance ID: %<ASMInstanceID>
  Terminator : Terminator
  Terminator1 : Terminator
  Terminator2 : Terminator
  Vectorize_Signals : Subsystem
  "[11:15]" : Selector  IndexOptions=Index vector (dialog)  Indices=[11:15]  OutputSizes=1
  "[1:5]" : Selector  IndexOptions=Index vector (dialog)  Indices=[1:5]  OutputSizes=1
  "[6:10]" : Selector  IndexOptions=Index vector (dialog)  Indices=[6:10]  OutputSizes=1
  Object_Custom_Values[] : Outport  VectorParamsAs1DForOutWhenUnconnected=off
  wires:
  CUSTOM_SENSOR_OUTPUT2/2 -> Vectorize_Signals/3(SensorOutput3)
  CUSTOM_SENSOR_OUTPUT1/2 -> Vectorize_Signals/2(SensorOutput2)
  Vectorize_Signals/1(Vectorized_Custom_Values) -> Object_Custom_Values[]/1
  CUSTOM_SENSOR_OUTPUT/2 -> Vectorize_Signals/1(SensorOutput1)
  CUSTOM_SENSOR_OUTPUT2/1 -> Terminator2/1
  CUSTOM_SENSOR_OUTPUT1/1 -> Terminator1/1
  CUSTOM_SENSOR_OUTPUT/1 -> Terminator/1
  "[6:10]"/1 -> CUSTOM_SENSOR_OUTPUT1/1
  TrafficObject_Type[]/1 -> "[11:15]"/1, "[6:10]"/1, "[1:5]"/1
  TrafficObject_Type_Data[]/1 -> CUSTOM_SENSOR_OUTPUT2/2, CUSTOM_SENSOR_OUTPUT1/2, CUSTOM_SENSOR_OUTPUT/2
  "[1:5]"/1 -> CUSTOM_SENSOR_OUTPUT/1
  "[11:15]"/1 -> CUSTOM_SENSOR_OUTPUT2/1

== system ASM_Traffic_MultiCore/Environment/Sensors/PlantModel/Object_Sensor_2D/ObjectData/Sensor4/ASMSignalCollector ==
  Object_Positions : Inport
  Object_Properties_Box : Inport  Port=2
  Object_Custom_Values : Inport  Port=3
  Bus Creator1 : BusCreator  Inputs=3
  Bus Selector : BusSelector  OutputSignals=Object_Positions
  Bus Selector1 : BusSelector  OutputSignals=Object_Properties_Box
  ASMSignalBus : Outport  VectorParamsAs1DForOutWhenUnconnected=off
  wires:
  Object_Positions/1 -> Bus Selector/1
  Object_Custom_Values/1 -> Bus Creator1/3
  Bus Creator1/1 -> ASMSignalBus/1  "ObjectData"
  Object_Properties_Box/1 -> Bus Selector1/1
  Bus Selector/1 -> Bus Creator1/1  "<Object_Positions>"
  Bus Selector1/1 -> Bus Creator1/2  "<Object_Properties_Box>"

== system ASM_Traffic_MultiCore/Environment/Sensors/PlantModel/Object_Sensor_2D/ObjectData/Sensor4/GetFellowPositionVector ==
  <FellowPositions> : Inport
  Bus Selector11 : BusSelector  OutputSignals=Pos_Fellows_MainPnt_CoorSys_E[x;y;z][m].Pos_x_Fellows[m],Pos_Fellows_MainPnt_CoorSys_E[x;y;z][m].Pos_y_Fellows[m],Pos_Fellows_MainPnt_CoorSys_E[x;y;z][m].Pos_z_Fellows[m],Angle_Fellows[x;y;z][deg].Angle_Roll_Fellows[deg],Angle_Fellows[x;y;z][deg].Angle_Pitch_Fellows[deg],Angle_Fellows[x;y;z][deg].Angle_Yaw_Fellows[deg]
  Mux1 : Mux  Inputs=3
  Mux2 : Mux  Inputs=3
  Pos_Fellows_MainPnt_CoorSys_E[x;y;z][m] : Outport  VectorParamsAs1DForOutWhenUnconnected=off
  Angle_Fellows[deg] : Outport  Port=2  VectorParamsAs1DForOutWhenUnconnected=off
  wires:
  Mux2/1 -> Pos_Fellows_MainPnt_CoorSys_E[x;y;z][m]/1  "Pos_Fellows_MainPnt_CoorSys_E[x;y;z][m]"
  Mux1/1 -> Angle_Fellows[deg]/1  "Pos_Fellows_MainPnt_CoorSys_E_vec"
  Bus Selector11/4 -> Mux1/1  "<Angle_Roll_Fellows[deg]>"
  Bus Selector11/1 -> Mux2/1  "<Pos_x_Fellows[m]>"
  Bus Selector11/2 -> Mux2/2  "<Pos_y_Fellows[m]>"
  Bus Selector11/6 -> Mux1/3  "<Angle_Yaw_Fellows[deg]>"
  Bus Selector11/5 -> Mux1/2  "<Angle_Pitch_Fellows[deg]>"
  <FellowPositions>/1 -> Bus Selector11/1
  Bus Selector11/3 -> Mux2/3  "<Pos_z_Fellows[m]>"

== system ASM_Traffic_MultiCore/Environment/Sensors/PlantModel/Object_Sensor_2D/ObjectData/Sensor4/Object_Custom_Values ==
  TrafficObject_Type[] : Inport
  TrafficObject_Type_Data[] : Inport  Port=2
  CUSTOM_SENSOR_OUTPUT : ASM_Traffic_lib/Sensors/Custom_Sensor/CUSTOM_SENSOR_OUTPUT  Tag=ASM_SUBCOMPONENT  ASMProperties=struct('Name','CUSTOM_SENSOR_OUTPUT','Version','5.0','Library','ASM_Traffic_lib')  ASMInstanceName=custom_sensor_output  ASMInstanceID=20
      settings: AttributesFormatString=Instance Name: %<ASMInstanceName>\nInstance ID: %<ASMInstanceID>
  CUSTOM_SENSOR_OUTPUT1 : ASM_Traffic_lib/Sensors/Custom_Sensor/CUSTOM_SENSOR_OUTPUT  Tag=ASM_SUBCOMPONENT  ASMProperties=struct('Name','CUSTOM_SENSOR_OUTPUT','Version','5.0','Library','ASM_Traffic_lib')  ASMInstanceName=custom_sensor_output  ASMInstanceID=21
      settings: AttributesFormatString=Instance Name: %<ASMInstanceName>\nInstance ID: %<ASMInstanceID>
  CUSTOM_SENSOR_OUTPUT2 : ASM_Traffic_lib/Sensors/Custom_Sensor/CUSTOM_SENSOR_OUTPUT  Tag=ASM_SUBCOMPONENT  ASMProperties=struct('Name','CUSTOM_SENSOR_OUTPUT','Version','5.0','Library','ASM_Traffic_lib')  ASMInstanceName=custom_sensor_output  ASMInstanceID=22
      settings: AttributesFormatString=Instance Name: %<ASMInstanceName>\nInstance ID: %<ASMInstanceID>
  Terminator : Terminator
  Terminator1 : Terminator
  Terminator2 : Terminator
  Vectorize_Signals : Subsystem
  "[11:15]" : Selector  IndexOptions=Index vector (dialog)  Indices=[11:15]  OutputSizes=1
  "[1:5]" : Selector  IndexOptions=Index vector (dialog)  Indices=[1:5]  OutputSizes=1
  "[6:10]" : Selector  IndexOptions=Index vector (dialog)  Indices=[6:10]  OutputSizes=1
  Object_Custom_Values[] : Outport  VectorParamsAs1DForOutWhenUnconnected=off
  wires:
  CUSTOM_SENSOR_OUTPUT2/2 -> Vectorize_Signals/3(SensorOutput3)
  CUSTOM_SENSOR_OUTPUT1/2 -> Vectorize_Signals/2(SensorOutput2)
  Vectorize_Signals/1(Vectorized_Custom_Values) -> Object_Custom_Values[]/1
  CUSTOM_SENSOR_OUTPUT/2 -> Vectorize_Signals/1(SensorOutput1)
  CUSTOM_SENSOR_OUTPUT2/1 -> Terminator2/1
  CUSTOM_SENSOR_OUTPUT1/1 -> Terminator1/1
  CUSTOM_SENSOR_OUTPUT/1 -> Terminator/1
  "[6:10]"/1 -> CUSTOM_SENSOR_OUTPUT1/1
  TrafficObject_Type[]/1 -> "[1:5]"/1, "[6:10]"/1, "[11:15]"/1
  TrafficObject_Type_Data[]/1 -> CUSTOM_SENSOR_OUTPUT2/2, CUSTOM_SENSOR_OUTPUT1/2, CUSTOM_SENSOR_OUTPUT/2
  "[1:5]"/1 -> CUSTOM_SENSOR_OUTPUT/1
  "[11:15]"/1 -> CUSTOM_SENSOR_OUTPUT2/1

== system ASM_Traffic_MultiCore/Environment/Sensors/PlantModel/Object_Sensor_2D/ObjectData/Sensor5/ASMSignalCollector ==
  Object_Positions : Inport
  Object_Properties_Box : Inport  Port=2
  Object_Custom_Values : Inport  Port=3
  Bus Creator1 : BusCreator  Inputs=3
  Bus Selector : BusSelector  OutputSignals=Object_Positions
  Bus Selector1 : BusSelector  OutputSignals=Object_Properties_Box
  ASMSignalBus : Outport  VectorParamsAs1DForOutWhenUnconnected=off
  wires:
  Object_Positions/1 -> Bus Selector/1
  Object_Custom_Values/1 -> Bus Creator1/3
  Bus Creator1/1 -> ASMSignalBus/1  "ObjectData"
  Object_Properties_Box/1 -> Bus Selector1/1
  Bus Selector/1 -> Bus Creator1/1  "<Object_Positions>"
  Bus Selector1/1 -> Bus Creator1/2  "<Object_Properties_Box>"

== system ASM_Traffic_MultiCore/Environment/Sensors/PlantModel/Object_Sensor_2D/ObjectData/Sensor5/GetFellowPositionVector ==
  <FellowPositions> : Inport
  Bus Selector11 : BusSelector  OutputSignals=Pos_Fellows_MainPnt_CoorSys_E[x;y;z][m].Pos_x_Fellows[m],Pos_Fellows_MainPnt_CoorSys_E[x;y;z][m].Pos_y_Fellows[m],Pos_Fellows_MainPnt_CoorSys_E[x;y;z][m].Pos_z_Fellows[m],Angle_Fellows[x;y;z][deg].Angle_Roll_Fellows[deg],Angle_Fellows[x;y;z][deg].Angle_Pitch_Fellows[deg],Angle_Fellows[x;y;z][deg].Angle_Yaw_Fellows[deg]
  Mux1 : Mux  Inputs=3
  Mux2 : Mux  Inputs=3
  Pos_Fellows_MainPnt_CoorSys_E[x;y;z][m] : Outport  VectorParamsAs1DForOutWhenUnconnected=off
  Angle_Fellows[deg] : Outport  Port=2  VectorParamsAs1DForOutWhenUnconnected=off
  wires:
  Mux2/1 -> Pos_Fellows_MainPnt_CoorSys_E[x;y;z][m]/1  "Pos_Fellows_MainPnt_CoorSys_E[x;y;z][m]"
  Mux1/1 -> Angle_Fellows[deg]/1  "Pos_Fellows_MainPnt_CoorSys_E_vec"
  Bus Selector11/4 -> Mux1/1  "<Angle_Roll_Fellows[deg]>"
  Bus Selector11/1 -> Mux2/1  "<Pos_x_Fellows[m]>"
  Bus Selector11/2 -> Mux2/2  "<Pos_y_Fellows[m]>"
  Bus Selector11/6 -> Mux1/3  "<Angle_Yaw_Fellows[deg]>"
  Bus Selector11/5 -> Mux1/2  "<Angle_Pitch_Fellows[deg]>"
  <FellowPositions>/1 -> Bus Selector11/1
  Bus Selector11/3 -> Mux2/3  "<Pos_z_Fellows[m]>"

== system ASM_Traffic_MultiCore/Environment/Sensors/PlantModel/Object_Sensor_2D/ObjectData/Sensor5/Object_Custom_Values ==
  TrafficObject_Type[] : Inport
  TrafficObject_Type_Data[] : Inport  Port=2
  CUSTOM_SENSOR_OUTPUT : ASM_Traffic_lib/Sensors/Custom_Sensor/CUSTOM_SENSOR_OUTPUT  Tag=ASM_SUBCOMPONENT  ASMProperties=struct('Name','CUSTOM_SENSOR_OUTPUT','Version','5.0','Library','ASM_Traffic_lib')  ASMInstanceName=custom_sensor_output  ASMInstanceID=23
      settings: AttributesFormatString=Instance Name: %<ASMInstanceName>\nInstance ID: %<ASMInstanceID>
  CUSTOM_SENSOR_OUTPUT1 : ASM_Traffic_lib/Sensors/Custom_Sensor/CUSTOM_SENSOR_OUTPUT  Tag=ASM_SUBCOMPONENT  ASMProperties=struct('Name','CUSTOM_SENSOR_OUTPUT','Version','5.0','Library','ASM_Traffic_lib')  ASMInstanceName=custom_sensor_output  ASMInstanceID=24
      settings: AttributesFormatString=Instance Name: %<ASMInstanceName>\nInstance ID: %<ASMInstanceID>
  CUSTOM_SENSOR_OUTPUT2 : ASM_Traffic_lib/Sensors/Custom_Sensor/CUSTOM_SENSOR_OUTPUT  Tag=ASM_SUBCOMPONENT  ASMProperties=struct('Name','CUSTOM_SENSOR_OUTPUT','Version','5.0','Library','ASM_Traffic_lib')  ASMInstanceName=custom_sensor_output  ASMInstanceID=25
      settings: AttributesFormatString=Instance Name: %<ASMInstanceName>\nInstance ID: %<ASMInstanceID>
  Terminator : Terminator
  Terminator1 : Terminator
  Terminator2 : Terminator
  Vectorize_Signals : Subsystem
  "[11:15]" : Selector  IndexOptions=Index vector (dialog)  Indices=[11:15]  OutputSizes=1
  "[1:5]" : Selector  IndexOptions=Index vector (dialog)  Indices=[1:5]  OutputSizes=1
  "[6:10]" : Selector  IndexOptions=Index vector (dialog)  Indices=[6:10]  OutputSizes=1
  Object_Custom_Values[] : Outport  VectorParamsAs1DForOutWhenUnconnected=off
  wires:
  "[11:15]"/1 -> CUSTOM_SENSOR_OUTPUT2/1
  "[1:5]"/1 -> CUSTOM_SENSOR_OUTPUT/1
  TrafficObject_Type_Data[]/1 -> CUSTOM_SENSOR_OUTPUT2/2, CUSTOM_SENSOR_OUTPUT1/2, CUSTOM_SENSOR_OUTPUT/2
  TrafficObject_Type[]/1 -> "[11:15]"/1, "[6:10]"/1, "[1:5]"/1
  "[6:10]"/1 -> CUSTOM_SENSOR_OUTPUT1/1
  CUSTOM_SENSOR_OUTPUT/1 -> Terminator/1
  CUSTOM_SENSOR_OUTPUT1/1 -> Terminator1/1
  CUSTOM_SENSOR_OUTPUT2/1 -> Terminator2/1
  CUSTOM_SENSOR_OUTPUT/2 -> Vectorize_Signals/1(SensorOutput1)
  Vectorize_Signals/1(Vectorized_Custom_Values) -> Object_Custom_Values[]/1
  CUSTOM_SENSOR_OUTPUT1/2 -> Vectorize_Signals/2(SensorOutput2)
  CUSTOM_SENSOR_OUTPUT2/2 -> Vectorize_Signals/3(SensorOutput3)

== system ASM_Traffic_MultiCore/Environment/Sensors/PlantModel/Object_Sensor_2D/ObjectData/Sensor6/ASMSignalCollector ==
  Object_Positions : Inport
  Object_Properties_Box : Inport  Port=2
  Object_Custom_Values : Inport  Port=3
  Bus Creator1 : BusCreator  Inputs=3
  Bus Selector : BusSelector  OutputSignals=Object_Positions
  Bus Selector1 : BusSelector  OutputSignals=Object_Properties_Box
  ASMSignalBus : Outport  VectorParamsAs1DForOutWhenUnconnected=off
  wires:
  Object_Positions/1 -> Bus Selector/1
  Object_Custom_Values/1 -> Bus Creator1/3
  Bus Creator1/1 -> ASMSignalBus/1  "ObjectData"
  Object_Properties_Box/1 -> Bus Selector1/1
  Bus Selector/1 -> Bus Creator1/1  "<Object_Positions>"
  Bus Selector1/1 -> Bus Creator1/2  "<Object_Properties_Box>"

== system ASM_Traffic_MultiCore/Environment/Sensors/PlantModel/Object_Sensor_2D/ObjectData/Sensor6/GetFellowPositionVector ==
  <FellowPositions> : Inport
  Bus Selector11 : BusSelector  OutputSignals=Pos_Fellows_MainPnt_CoorSys_E[x;y;z][m].Pos_x_Fellows[m],Pos_Fellows_MainPnt_CoorSys_E[x;y;z][m].Pos_y_Fellows[m],Pos_Fellows_MainPnt_CoorSys_E[x;y;z][m].Pos_z_Fellows[m],Angle_Fellows[x;y;z][deg].Angle_Roll_Fellows[deg],Angle_Fellows[x;y;z][deg].Angle_Pitch_Fellows[deg],Angle_Fellows[x;y;z][deg].Angle_Yaw_Fellows[deg]
  Mux1 : Mux  Inputs=3
  Mux2 : Mux  Inputs=3
  Pos_Fellows_MainPnt_CoorSys_E[x;y;z][m] : Outport  VectorParamsAs1DForOutWhenUnconnected=off
  Angle_Fellows[deg] : Outport  Port=2  VectorParamsAs1DForOutWhenUnconnected=off
  wires:
  Mux2/1 -> Pos_Fellows_MainPnt_CoorSys_E[x;y;z][m]/1  "Pos_Fellows_MainPnt_CoorSys_E[x;y;z][m]"
  Mux1/1 -> Angle_Fellows[deg]/1  "Pos_Fellows_MainPnt_CoorSys_E_vec"
  Bus Selector11/4 -> Mux1/1  "<Angle_Roll_Fellows[deg]>"
  Bus Selector11/1 -> Mux2/1  "<Pos_x_Fellows[m]>"
  Bus Selector11/2 -> Mux2/2  "<Pos_y_Fellows[m]>"
  Bus Selector11/6 -> Mux1/3  "<Angle_Yaw_Fellows[deg]>"
  Bus Selector11/5 -> Mux1/2  "<Angle_Pitch_Fellows[deg]>"
  <FellowPositions>/1 -> Bus Selector11/1
  Bus Selector11/3 -> Mux2/3  "<Pos_z_Fellows[m]>"
